simulink model "ece308hw3simu"  (R2025a)
settings: Solver=ode4  StartTime=0.0  StopTime=25  FixedStep=0.002  RelTol=1e-3
undefined symbols (not defined in the file or in its folder): a, b, Kc, wcf, wf, z, zcf
settings Model: Creator=jaldana  LastModifiedBy=jaldana

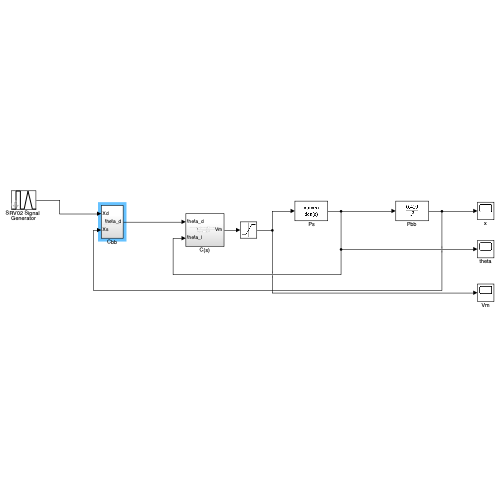
[thumbnail: Simulink's stored preview of the top-level diagram]
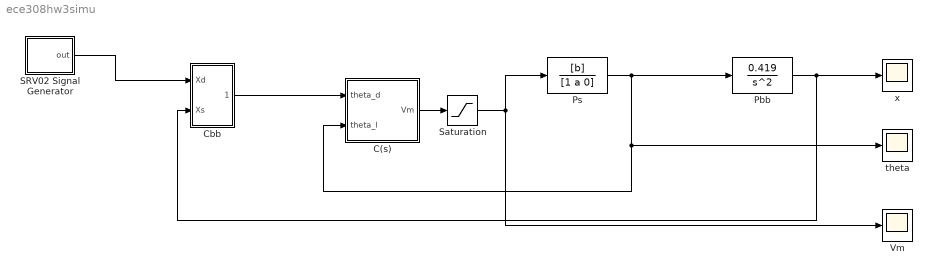
== system ece308hw3simu ==
  " Ps" : TransferFcn  Numerator=[b]  Denominator=[1 a 0]
  C(s) : Subsystem
  Cbb : Subsystem
  Pbb : TransferFcn  Numerator=[0.419]  Denominator=[1 0 0]
  SRV02 Signal Generator : Subsystem  mask(QET Signal Generator){sig_type=square, a=0.05, f=0.05}
      mask prompts: sig_type "Signal Type"; a "Amplitude"; f "Frequency (Hz)"
      mask help: Generates a square, triangular, or sinusoidal waveform of a specified amplitude and frequency.
      mask Help: Choose the type of signal to be generated from the drop-down "Signal Type" box. Enter the amplitude and the frequency desired for the signal. Note: frequency is in Hertz.
      mask TypeOptions sig_type: square | triangle | sine
      mask Display: plot([0 1 1 2 2 3 4 5 6], [-1 -1 1 1 -1 -1 1 -1 -1])
  Saturation : Saturate  UpperLimit=10  LowerLimit=-10
  Vm : Scope
      settings: ActiveDisplayYMinimum=-1  ActiveDisplayYMaximum=1  DataLoggingVariableName=ScopeData2
  theta : Scope
      settings: ActiveDisplayYMinimum=-1  ActiveDisplayYMaximum=1
  x : Scope
      settings: ActiveDisplayYMinimum=-6.5329281552990439  ActiveDisplayYMaximum=9.4102458514182974
  wires:
  " Ps"/1 -> theta/1, C(s)/2(theta_l), Pbb/1
  SRV02 Signal Generator/1(out) -> Cbb/1(Xd)
  Pbb/1 -> Cbb/2(Xs), x/1
  Cbb/1(theta_d) -> C(s)/1(theta_d)
  C(s)/1(Vm) -> Saturation/1
  Saturation/1 -> Vm/1, " Ps"/1

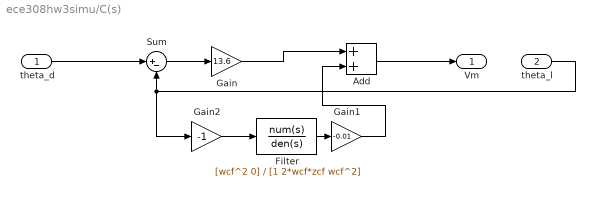
== system ece308hw3simu/C(s) ==
  theta_d : Inport
  theta_l : Inport  Port=2
  Add : Sum
  Filter : TransferFcn  Numerator=[wcf^2 0]  Denominator=[1 2*wcf*zcf wcf^2]
  Gain : Gain  Gain=13.6
  Gain1 : Gain  Gain=-0.01
  Gain2 : Gain  Gain=-1
  Sum : Sum  Inputs=|+-
  Vm : Outport
  wires:
  Add/1 -> Vm/1
  Gain2/1 -> Filter/1
  Sum/1 -> Gain/1
  Filter/1 -> Gain1/1
  theta_l/1 -> Gain2/1, Sum/2
  Gain1/1 -> Add/2
  theta_d/1 -> Sum/1
  Gain/1 -> Add/1

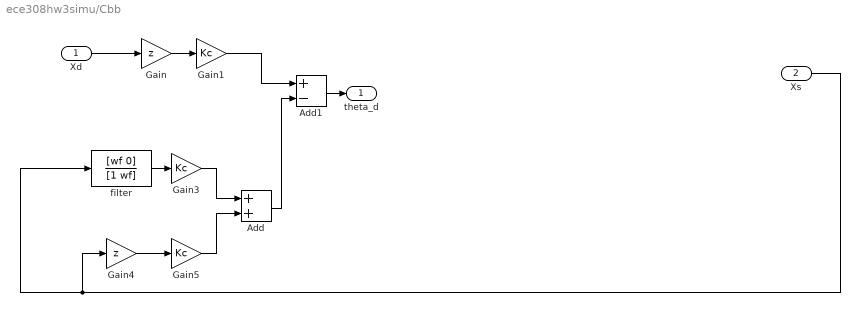
== system ece308hw3simu/Cbb ==
  Xd : Inport
  Xs : Inport  Port=2
  " filter" : TransferFcn  Numerator=[wf 0]  Denominator=[1 wf]
  Add : Sum
  Add1 : Sum  Inputs=+-
  Gain : Gain  Gain=z
  Gain1 : Gain  Gain=Kc
  Gain3 : Gain  Gain=Kc
  Gain4 : Gain  Gain=z
  Gain5 : Gain  Gain=Kc
  theta_d : Outport
  wires:
  Gain/1 -> Gain1/1
  Add1/1 -> theta_d/1
  " filter"/1 -> Gain3/1
  Add/1 -> Add1/2
  Gain5/1 -> Add/2
  Xd/1 -> Gain/1
  Gain4/1 -> Gain5/1
  Gain1/1 -> Add1/1
  Gain3/1 -> Add/1
  Xs/1 -> Gain4/1, " filter"/1

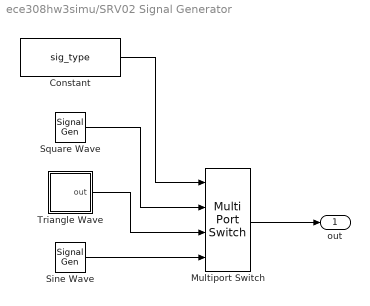
== system ece308hw3simu/SRV02 Signal Generator ==
  Constant : Constant  Value=sig_type
  Multiport Switch : MultiPortSwitch  SaturateOnIntegerOverflow=off  InputSameDT=off
  Sine Wave : SignalGenerator  Amplitude=a  Frequency=f
  Square Wave : SignalGenerator  WaveForm=square  Amplitude=a  Frequency=f
  Triangle Wave : Subsystem
  out : Outport
  wires:
  Square Wave/1 -> Multiport Switch/2
  Triangle Wave/1(out) -> Multiport Switch/3
  Sine Wave/1 -> Multiport Switch/4
  Multiport Switch/1 -> out/1
  Constant/1 -> Multiport Switch/1

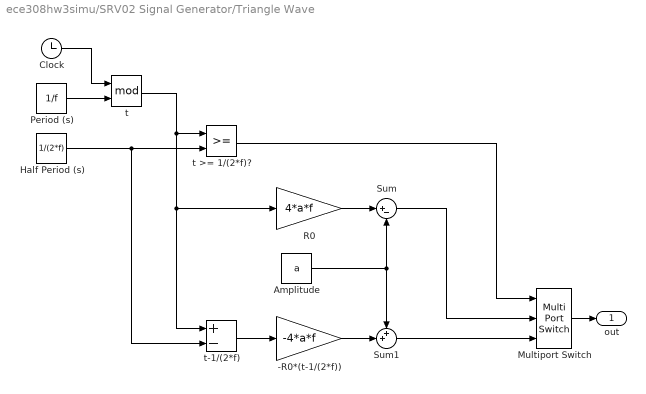
== system ece308hw3simu/SRV02 Signal Generator/Triangle Wave ==
  -R0*(t-1/(2*f)) : Gain  Gain=-4*a*f
  Amplitude : Constant  Value=a
  Clock : Clock
  Half Period (s) : Constant  Value=1/(2*f)
  Multiport Switch : MultiPortSwitch  DataPortOrder=Zero-based contiguous  Inputs=2  zeroidx=on  SaturateOnIntegerOverflow=off  InputSameDT=off
  Period (s) : Constant  Value=1/f
  R0 : Gain  Gain=4*a*f
  Sum : Sum  Inputs=|+-
  Sum1 : Sum  Inputs=++|
  t : Math  Operator=mod  SignedPower=on
  t >= 1/(2*f)? : RelationalOperator  OutDataTypeStr=boolean  InputSameDT=off
  t-1/(2*f) : Sum  Inputs=+-
  out : Outport
  wires:
  Sum1/1 -> Multiport Switch/3
  Sum/1 -> Multiport Switch/2
  t >= 1/(2*f)?/1 -> Multiport Switch/1
  -R0*(t-1/(2*f))/1 -> Sum1/2
  Amplitude/1 -> Sum1/1, Sum/2
  R0/1 -> Sum/1
  t-1/(2*f)/1 -> -R0*(t-1/(2*f))/1
  Half Period (s)/1 -> t-1/(2*f)/2, t >= 1/(2*f)?/2
  t/1 -> t-1/(2*f)/1, R0/1, t >= 1/(2*f)?/1
  Period (s)/1 -> t/2
  Clock/1 -> t/1
  Multiport Switch/1 -> out/1
